simulink model "ev_pmsm_foc_drive"  (R2025b)
settings: Solver=ode4  StartTime=0.0  StopTime=0.25  FixedStep=1e-4  RelTol=1e-3
settings Model: Creator=user  LastModifiedBy=user

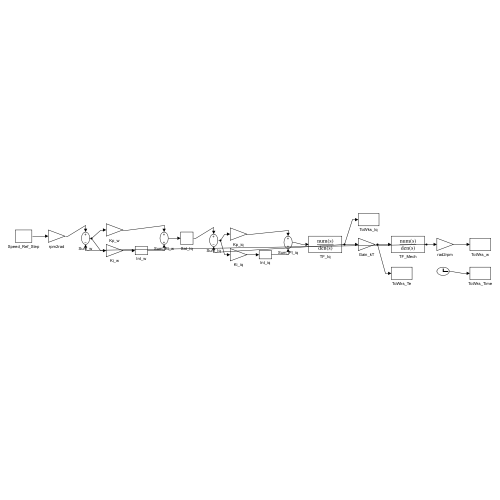
[thumbnail: Simulink's stored preview of the top-level diagram]
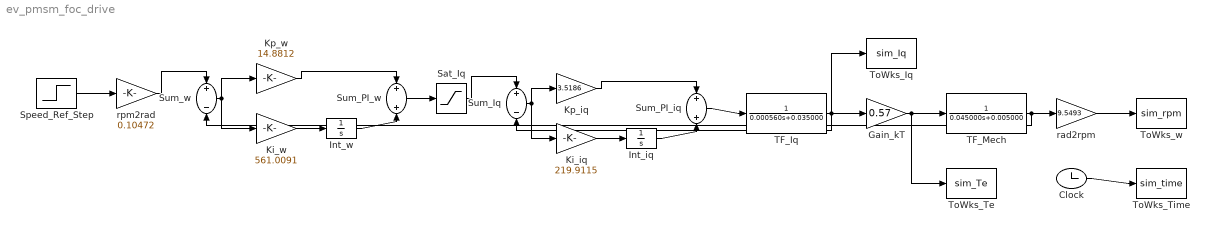
== system ev_pmsm_foc_drive ==
  Clock : Clock
  Gain_kT : Gain  Gain=0.57
  Int_iq : Integrator
  Int_w : Integrator
  Ki_iq : Gain  Gain=219.9115
  Ki_w : Gain  Gain=561.0091
  Kp_iq : Gain  Gain=3.5186
  Kp_w : Gain  Gain=14.8812
  Sat_Iq : Saturate  UpperLimit=250  LowerLimit=-250
  Speed_Ref_Step : Step  Time=0.02  After=1500  SampleTime=0
  Sum_Iq : Sum  Inputs=+-
  Sum_PI_iq : Sum
  Sum_PI_w : Sum
  Sum_w : Sum  Inputs=+-
  TF_Iq : TransferFcn  Denominator=[0.000560 0.035000]
  TF_Mech : TransferFcn  Denominator=[0.045000 0.005000]
  ToWks_Iq : ToWorkspace  VariableName=sim_Iq  SampleTime=-1
  ToWks_Te : ToWorkspace  VariableName=sim_Te  SampleTime=-1
  ToWks_Time : ToWorkspace  VariableName=sim_time  SampleTime=-1
  ToWks_w : ToWorkspace  VariableName=sim_rpm  SampleTime=-1
  rad2rpm : Gain  Gain=9.5493
  rpm2rad : Gain  Gain=0.10472
  wires:
  Speed_Ref_Step/1 -> rpm2rad/1
  rpm2rad/1 -> Sum_w/1
  Sum_w/1 -> Kp_w/1, Ki_w/1
  Ki_w/1 -> Int_w/1
  Kp_w/1 -> Sum_PI_w/1
  Int_w/1 -> Sum_PI_w/2
  Sum_PI_w/1 -> Sat_Iq/1
  Sat_Iq/1 -> Sum_Iq/1
  Sum_Iq/1 -> Kp_iq/1, Ki_iq/1
  Ki_iq/1 -> Int_iq/1
  Kp_iq/1 -> Sum_PI_iq/1
  Int_iq/1 -> Sum_PI_iq/2
  Sum_PI_iq/1 -> TF_Iq/1
  TF_Iq/1 -> Sum_Iq/2, Gain_kT/1, ToWks_Iq/1
  Gain_kT/1 -> TF_Mech/1, ToWks_Te/1
  TF_Mech/1 -> Sum_w/2, rad2rpm/1
  rad2rpm/1 -> ToWks_w/1
  Clock/1 -> ToWks_Time/1
